simulink model "heli_q8lab2"  (R2020b)
settings: Solver=ode1  StartTime=0.0  StopTime=inf  FixedStep=0.002  RelTol=1e-3  EnableMultiTasking=on
PostLoadFcn:
  | qc_set_target_type(getConfigSet(bdroot, 'QUARC Default Target Configuration'));
values from neighbouring files (symbols this model uses):
  F = [0 0; 0 0]    [init_heli_3_10lab2integral.m]    (also in init_heli_3_10lab2nointegral.m = [K(1, 1) K(1, 3))
  Joystick_gain_x = 1    [init_heli_3_10lab2integral.m]    (also in init_heli_3_10lab2nointegral.m)
  Joystick_gain_y = -1    [init_heli_3_10lab2integral.m]    (also in init_heli_3_10lab2nointegral.m)
  K_pd = -(lambda_1 + lambda_2)/K1    [init_heli_3_10lab2integral.m]    (also in init_heli_3_10lab2nointegral.m)
  K_pp = (lambda_1*lambda_2)/K1    [init_heli_3_10lab2integral.m]    (also in init_heli_3_10lab2nointegral.m)
undefined symbols (not defined in the file or in its folder): HIL, K, qc_get_step_size
libraries: quarc_library x4
settings Model: SimulationMode=external  ExtModeTrigDuration=5000  Creator=Rchan  LastModifiedBy=arnstein
settings SolverCC: PositivePriorityOrder=on
settings DataIOCC: LimitDataPoints=on  SaveFormat=Array  SignalLoggingSaveFormat=ModelDataLogs  ReturnWorkspaceOutputs=off
settings OptimizationCC: ExpressionDepthLimit=2147483647  InitFltsAndDblsToZero=on  LifeSpan=inf
settings DebuggingCC: SaveWithParameterizedLinksMsg=none  UnderspecifiedInitializationDetection=Classic  MergeDetectMultiDrivingBlocksExec=none  SolverPrmCheckMsg=warning  MultiTaskDSMMsg=warning  MultiTaskCondExecSysMsg=none  FcnCallInpInsideContextMsg=warning  AllowSymbolicDim=off  StateNameClashWarn=warning  SFUnexpectedBacktrackingDiag=warning  SFNoUnconditionalDefaultTransitionDiag=warning  SFExecutionAtInitializationDiag=none  ArithmeticOperatorsInVariantConditions=warning
settings HardwareCC: ProdBitPerPointer=32  ProdBitPerSizeT=32  ProdBitPerPtrDiffT=32  ProdLargestAtomicFloat=None  ProdIntDivRoundTo=Undefined  ProdEndianess=Unspecified  ProdWordSize=32  ProdHWDeviceType=32-bit Generic
settings ModelReferenceCC: PropagateSignalLabelsOutOfModel=off
settings SFSimCC: SimUseLocalCustomCode=off  CustomCodeUndefinedFunction=UseInterfaceOnly
settings RTWCC: Description=QUARC Win64 Target  SystemTargetFile=quarc_win64.tlc  TemplateMakefile=quarc_default_tmf  RTWUseLocalCustomCode=off
settings CodeAppCC: StateflowObjectComments=on
settings GRTTargetCC: TargetLangStandard=C89/C90 (ANSI)  ParMdlRefBuildCompliant=off  CompOptLevelCompliant=off  CombineOutputUpdateFcns=off  MatFileLogging=off  GRTInterface=on  UseToolchainInfoCompliant=off  ExtMode=on  ExtModeMexFile=quarc_comm
settings ConfigComp: CovMetricSettings=de  CovSaveCumulativeToWorkspaceVar=on  CovSaveSingleToWorkspaceVar=on  CovExternalEMLEnable=off  CovSFcnEnable=off  CovBoundaryAbsTol=1.0e-5

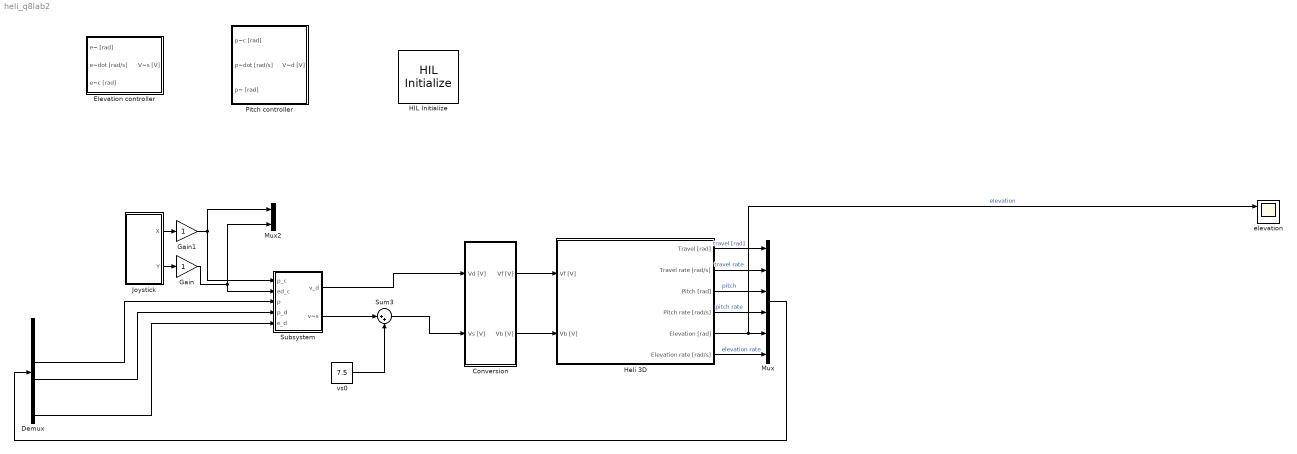
== system heli_q8lab2 ==
  Conversion : Subsystem
  Demux : Demux  Outputs=6
  Elevation controller : Subsystem
  Gain : Gain
  Gain1 : Gain
  HIL Initialize : quarc_library/Data Acquisition/Generic/Configuration/HIL Initialize  Priority=-99  object_name=HIL-1  board_type=q8_usb  board_number=0  board_options=update_rate=normal;decimation=1  exclusive=off  active=off  hardware_clocks=[0:2]  clock_modes=[]  initial_clock_frequencies=[]  set_clock_params_at_start=off  set_clock_params_at_switch_in=off  set_clock_frequencies_at_start=off  set_clock_frequencies_at_switch_in=off  analog_input_channels=[0:7]  analog_input_configurations=[]  analog_input_maximums=10  analog_input_minimums=-10  set_analog_input_params_at_start=on  set_analog_input_params_at_switch_in=off  analog_output_channels=[0:7]  analog_output_maximums=10  analog_output_minimums=-10  initial_analog_outputs=[0]  final_analog_outputs=[0]  watchdog_analog_outputs=0  set_analog_output_params_at_start=on  set_analog_output_params_at_switch_in=off  set_analog_outputs_at_start=on  set_analog_outputs_at_switch_in=off  set_analog_outputs_at_terminate=on  set_analog_outputs_at_switch_out=off  set_analog_outputs_on_watchdog=off  digital_input_channels=[]  digital_output_channels=[]  digital_output_configuration=[]  initial_digital_outputs=[1]  final_digital_outputs=[1]  watchdog_digital_outputs=[1]  set_digital_output_params_at_start=off  set_digital_output_params_at_switch_in=off  set_digital_outputs_at_start=on  set_digital_outputs_at_switch_in=off  set_digital_outputs_at_terminate=on  set_digital_outputs_at_switch_out=off  set_digital_outputs_on_watchdog=off  encoder_channels=[0:7]  quadrature=[4]  encoder_filter_frequency=[]  initial_encoder_counts=[0]  set_encoder_params_at_start=on  set_encoder_params_at_switch_in=off  set_encoder_counts_at_start=on  set_encoder_counts_at_switch_in=off  pwm_channels=[0:7]  pwm_modes=0  pwm_frequency=99.532799999999995e6/4095  pwm_configuration=[0]  pwm_alignment=[0]  pwm_polarity=[1]  pwm_leading_deadband=[0]  pwm_trailing_deadband=[0]  initial_pwm_outputs=[0]  final_pwm_outputs=[0]  watchdog_pwm_outputs=[0]  set_pwm_params_at_start=on  set_pwm_params_at_switch_in=off  set_pwm_outputs_at_start=on  set_pwm_outputs_at_switch_in=off  set_pwm_outputs_at_terminate=on  set_pwm_outputs_at_switch_out=off  set_pwm_outputs_on_watchdog=off  other_output_channels=[]  initial_other_outputs=[]  final_other_outputs=[]  watchdog_other_outputs=[]  set_other_outputs_at_start=off  set_other_outputs_at_switch_in=off  set_other_outputs_at_terminate=off  set_other_outputs_at_switch_out=off  set_other_outputs_on_watchdog=off
  Heli 3D : Subsystem
  Joystick : Subsystem
  Mux : Mux  Inputs=6
  Mux2 : Mux  Inputs=2
  Pitch controller : Subsystem
  Subsystem : Subsystem
  Sum3 : Sum  Inputs=|++
  elevation : Scope  NumInputPorts=2
  vs0 : Constant  Value=7.5
  wires:
  Conversion/2(Vb [V]) -> Heli 3D/2(Vb [V])
  Conversion/1(Vf [V]) -> Heli 3D/1(Vf [V])
  Heli 3D/1(Travel [rad]) -> Mux/1  "travel [rad]"
  Heli 3D/2(Travel rate [rad/s]) -> Mux/2  "travel rate"
  Heli 3D/3(Pitch [rad]) -> Mux/3  "pitch"
  Heli 3D/4(Pitch rate [rad/s]) -> Mux/4  "pitch rate"
  Heli 3D/5(Elevation [rad]) -> elevation/1, Mux/5  "elevation"
  Heli 3D/6(Elevation rate [rad/s]) -> Mux/6  "elevation rate"
  Joystick/1(X) -> Gain1/1
  Joystick/2(Y) -> Gain/1
  Gain/1 -> Mux2/2, Subsystem/2(ed_c)
  Gain1/1 -> Mux2/1, Subsystem/1(p_c)
  Subsystem/1(v_d) -> Conversion/1(Vd [V])
  Subsystem/2(v~s) -> Sum3/1
  Sum3/1 -> Conversion/2(Vs [V])
  vs0/1 -> Sum3/2
  Demux/3 -> Subsystem/3(p)
  Demux/4 -> Subsystem/4(p_d)
  Demux/6 -> Subsystem/5(e_d)
  Mux/1 -> Demux/1

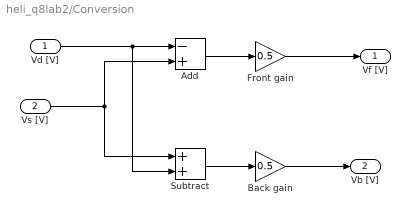
== system heli_q8lab2/Conversion ==
  Vd [V] : Inport
  Vs [V] : Inport  Port=2
  Add : Sum  Inputs=-+
  Back gain : Gain  Gain=0.5
  Front gain : Gain  Gain=0.5
  Subtract : Sum
  Vf [V] : Outport
  Vb [V] : Outport  Port=2
  wires:
  Vd [V]/1 -> Subtract/2, Add/1
  Vs [V]/1 -> Subtract/1, Add/2
  Subtract/1 -> Back gain/1
  Back gain/1 -> Vb [V]/1
  Add/1 -> Front gain/1
  Front gain/1 -> Vf [V]/1

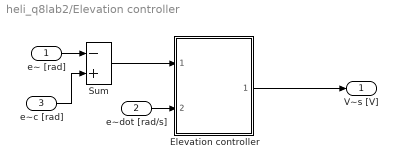
== system heli_q8lab2/Elevation controller ==
  e~ [rad] : Inport
  e~dot [rad/s] : Inport  Port=2
  e~c [rad] : Inport  Port=3
  Elevation controller : Subsystem
  Sum : Sum  Inputs=-+  InputSameDT=on  SaturateOnIntegerOverflow=on  OutDataTypeStr=Inherit: Same as first input
  V~s [V] : Outport  InitialOutput=0
  wires:
  Sum/1 -> Elevation controller/1(e~ [rad])
  Elevation controller/1(V~_s [V]) -> V~s [V]/1
  e~ [rad]/1 -> Sum/1
  e~dot [rad/s]/1 -> Elevation controller/2(e~_dot [rad/s])
  e~c [rad]/1 -> Sum/2

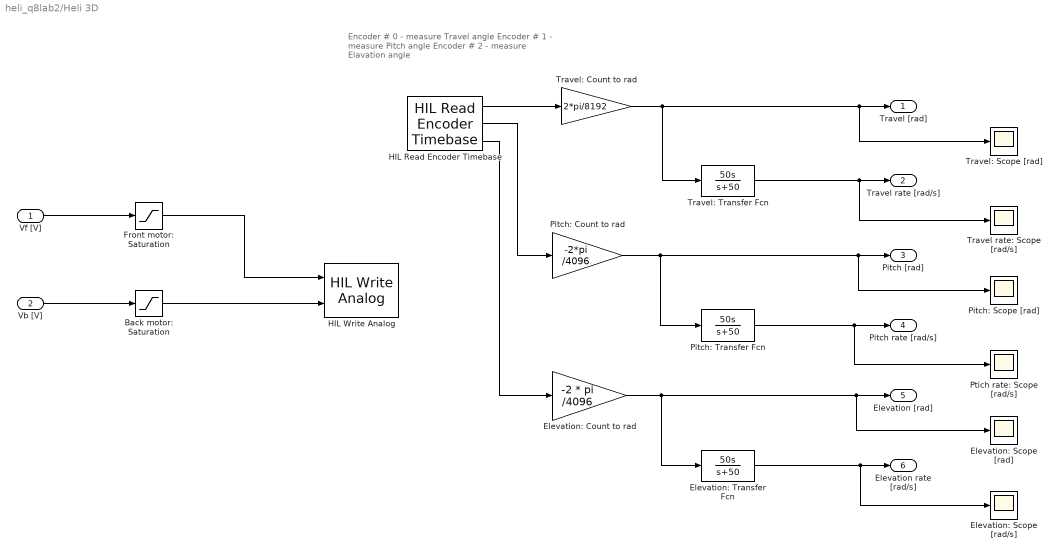
== system heli_q8lab2/Heli 3D ==
  note: Encoder # 0 - measure Travel angle
      | Encoder # 1 - measure Pitch angle
      | Encoder # 2 - measure Elavation angle
  Vf [V] : Inport
  Vb [V] : Inport  Port=2
  Back motor: Saturation : Saturate  UpperLimit=5  LowerLimit=-5
  Elevation: Count to rad : Gain  Gain=-2 * pi /4096
  Elevation: Scope [rad/s] : Scope
  Elevation: Scope [rad] : Scope
  Elevation: Transfer Fcn : TransferFcn  Numerator=[50 0]  Denominator=[1 50]
  Front motor: Saturation : Saturate  UpperLimit=5  LowerLimit=-5
  HIL Read Encoder Timebase : quarc_library/Data Acquisition/Generic/Timebases/HIL Read Encoder Timebase  object_name=HIL-1  clock=0  channels=[0:2]  active=on  vector_output=off  data_type_mode=Inherit via back propagation  data_type=double  overflow_mode=Error on overflow  samples_in_buffer=max(ceil(1/qc_get_step_size), 1)
  HIL Write Analog : quarc_library/Data Acquisition/Generic/Immediate I//O/HIL Write Analog  object_name=HIL-1  channels=[0:1]  sample_time=-1  active=off  vector_input=off
  Pitch: Count to rad : Gain  Gain=-2*pi /4096
  Pitch: Scope [rad] : Scope
  Pitch: Transfer Fcn : TransferFcn  Numerator=[50 0]  Denominator=[1 50]
  Ptich rate: Scope [rad/s] : Scope
  Travel rate: Scope [rad/s] : Scope
  Travel: Count to rad : Gain  Gain=2*pi/8192
  Travel: Scope [rad] : Scope
  Travel: Transfer Fcn : TransferFcn  Numerator=[50 0]  Denominator=[1 50]
  Travel [rad] : Outport
  Travel rate [rad/s] : Outport  Port=2
  Pitch [rad] : Outport  Port=3
  Pitch rate [rad/s] : Outport  Port=4
  Elevation [rad] : Outport  Port=5
  Elevation rate [rad/s] : Outport  Port=6
  wires:
  HIL Read Encoder Timebase/1 -> Travel: Count to rad/1
  HIL Read Encoder Timebase/2 -> Pitch: Count to rad/1
  HIL Read Encoder Timebase/3 -> Elevation: Count to rad/1
  Travel: Count to rad/1 -> Travel: Scope [rad]/1, Travel [rad]/1, Travel: Transfer Fcn/1
  Travel: Transfer Fcn/1 -> Travel rate: Scope [rad/s]/1, Travel rate [rad/s]/1
  Pitch: Count to rad/1 -> Pitch: Transfer Fcn/1, Pitch: Scope [rad]/1, Pitch [rad]/1
  Pitch: Transfer Fcn/1 -> Ptich rate: Scope [rad/s]/1, Pitch rate [rad/s]/1
  Elevation: Count to rad/1 -> Elevation: Transfer Fcn/1, Elevation: Scope [rad]/1, Elevation [rad]/1
  Elevation: Transfer Fcn/1 -> Elevation: Scope [rad/s]/1, Elevation rate [rad/s]/1
  Vf [V]/1 -> Front motor: Saturation/1
  Vb [V]/1 -> Back motor: Saturation/1
  Front motor: Saturation/1 -> HIL Write Analog/1
  Back motor: Saturation/1 -> HIL Write Analog/2

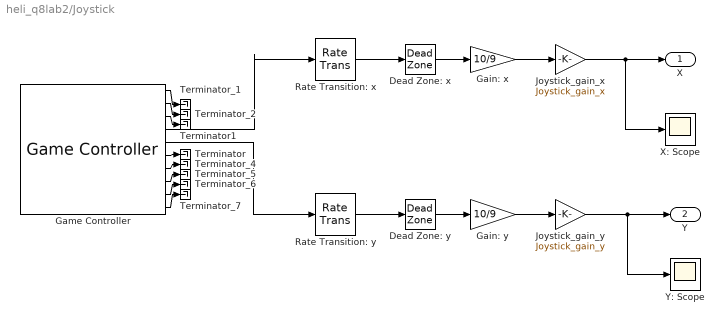
== system heli_q8lab2/Joystick ==
  Dead Zone: x : DeadZone  LowerValue=-0.1  UpperValue=0.1  SaturateOnIntegerOverflow=on
  Dead Zone: y : DeadZone  LowerValue=-0.1  UpperValue=0.1  SaturateOnIntegerOverflow=on
  Gain: x : Gain  Gain=10/9
  Gain: y : Gain  Gain=10/9
  Game Controller : quarc_library/Devices/Peripherals/Target/Game Controller  controller=1  buffer_size=12  deadzone=[]  saturation=[]  sample_time=max(qc_get_step_size, 0.01)  auto_center=off  enabled=on
      settings: SourceProductName=QUARC Targets
  Joystick_gain_x : Gain  Gain=Joystick_gain_x
  Joystick_gain_y : Gain  Gain=Joystick_gain_y
  Rate Transition: x : RateTransition
  Rate Transition: y : RateTransition
  Terminator : Terminator
  Terminator1 : Terminator
  Terminator_{1..2,4..7} (6 alike) : Terminator
  X: Scope : Scope
  Y: Scope : Scope
  X : Outport
  Y : Outport  Port=2
  wires:
  Rate Transition: y/1 -> Dead Zone: y/1
  Rate Transition: x/1 -> Dead Zone: x/1
  Game Controller/5 -> Rate Transition: y/1
  Game Controller/4 -> Rate Transition: x/1
  Game Controller/1 -> Terminator_1/1
  Game Controller/2 -> Terminator_2/1
  Game Controller/7 -> Terminator_4/1
  Game Controller/8 -> Terminator_5/1
  Game Controller/9 -> Terminator_6/1
  Game Controller/10 -> Terminator_7/1
  Game Controller/3 -> Terminator1/1
  Game Controller/6 -> Terminator/1
  Dead Zone: x/1 -> Gain: x/1
  Dead Zone: y/1 -> Gain: y/1
  Gain: x/1 -> Joystick_gain_x/1
  Gain: y/1 -> Joystick_gain_y/1
  Joystick_gain_x/1 -> X/1, X: Scope/1
  Joystick_gain_y/1 -> Y: Scope/1, Y/1

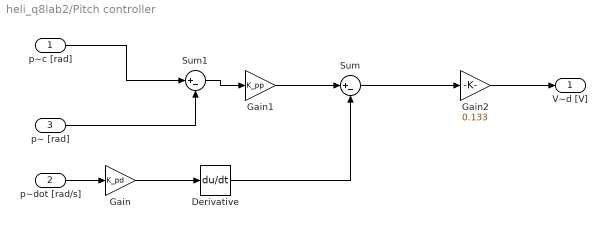
== system heli_q8lab2/Pitch controller ==
  p~c [rad] : Inport
  p~dot [rad/s] : Inport  Port=2
  p~ [rad] : Inport  Port=3
  Derivative : Derivative
  Gain : Gain  Gain=K_pd
  Gain1 : Gain  Gain=K_pp
  Gain2 : Gain  Gain=0.133
  Sum : Sum  Inputs=|+-
  Sum1 : Sum  Inputs=|+-
  V~d [V] : Outport  InitialOutput=0
  wires:
  p~dot [rad/s]/1 -> Gain/1
  Gain/1 -> Derivative/1
  Derivative/1 -> Sum/2
  p~c [rad]/1 -> Sum1/1
  p~ [rad]/1 -> Sum1/2
  Sum1/1 -> Gain1/1
  Gain1/1 -> Sum/1
  Sum/1 -> Gain2/1
  Gain2/1 -> V~d [V]/1

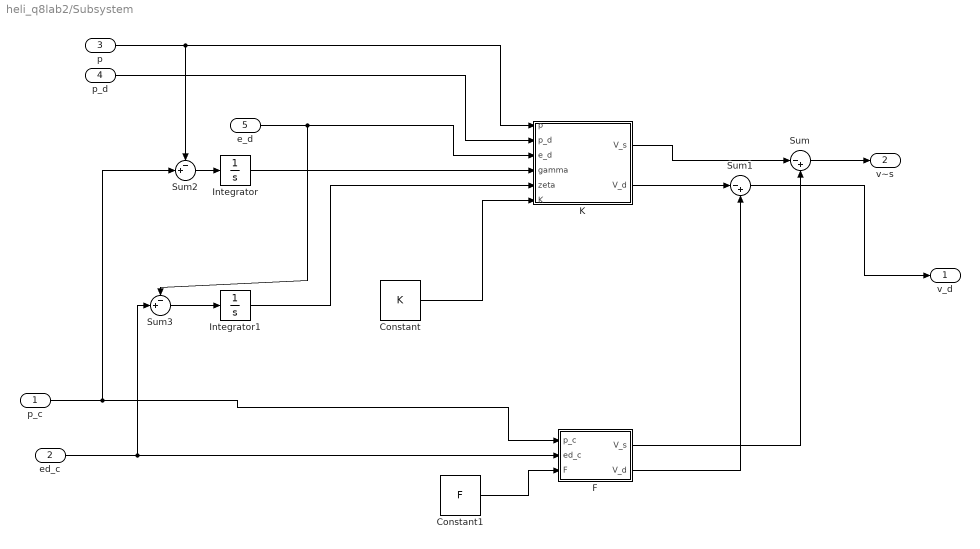
== system heli_q8lab2/Subsystem ==
  p_c : Inport
  ed_c : Inport  Port=2
  p : Inport  Port=3
  p_d : Inport  Port=4
  e_d : Inport  Port=5
  Constant : Constant  Value=K
  Constant1 : Constant  Value=F
  F : MATLAB Function  TreatAsAtomicUnit=on
  Integrator : Integrator
  Integrator1 : Integrator
  K : MATLAB Function  TreatAsAtomicUnit=on
  Sum : Sum  Inputs=|-+
  Sum1 : Sum  Inputs=|-+
  Sum2 : Sum  Inputs=-+|
  Sum3 : Sum  Inputs=-+|
  v_d : Outport
  v~s : Outport  Port=2
  wires:
  p/1 -> Sum2/1, K/1(p)
  p_d/1 -> K/2(p_d)
  e_d/1 -> Sum3/1, K/3(e_d)
  Constant/1 -> K/6(K)
  Constant1/1 -> F/3(F)
  p_c/1 -> Sum2/2, F/1(p_c)
  ed_c/1 -> Sum3/2, F/2(ed_c)
  K/1(V_s) -> Sum/1
  Sum/1 -> v~s/1
  K/2(V_d) -> Sum1/1
  F/1(V_s) -> Sum/2
  F/2(V_d) -> Sum1/2
  Sum1/1 -> v_d/1
  Integrator/1 -> K/4(gamma)
  Integrator1/1 -> K/5(zeta)
  Sum2/1 -> Integrator/1
  Sum3/1 -> Integrator1/1

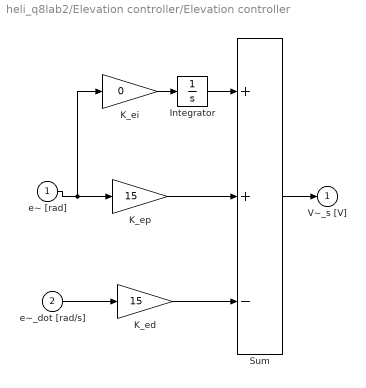
== system heli_q8lab2/Elevation controller/Elevation controller ==
  e~ [rad] : Inport
  e~_dot [rad/s] : Inport  Port=2
  Integrator : Integrator  LimitOutput=on
  K_ed : Gain  Gain=15  SaturateOnIntegerOverflow=on  OutDataTypeStr=Inherit: Same as input  ParamDataTypeStr=Inherit: Same as input
  K_ei : Gain  Gain=0  SaturateOnIntegerOverflow=on  OutDataTypeStr=Inherit: Same as input  ParamDataTypeStr=Inherit: Same as input
  K_ep : Gain  Gain=15  SaturateOnIntegerOverflow=on  OutDataTypeStr=Inherit: Same as input  ParamDataTypeStr=Inherit: Same as input
  Sum : Sum  Inputs=++-  InputSameDT=on  SaturateOnIntegerOverflow=on  OutDataTypeStr=Inherit: Same as first input
  V~_s [V] : Outport  InitialOutput=0
  wires:
  K_ei/1 -> Integrator/1
  Integrator/1 -> Sum/1
  Sum/1 -> V~_s [V]/1
  e~_dot [rad/s]/1 -> K_ed/1
  K_ed/1 -> Sum/3
  K_ep/1 -> Sum/2
  e~ [rad]/1 -> K_ep/1, K_ei/1

== matlab function heli_q8lab2/Subsystem/F ==
  data: p_c input; V_s output; V_d output; ed_c input; F input
function [V_s, V_d] = fcn(p_c, ed_c, F)
M = (F*[p_c, ed_c].');
V_s = M(1, :);
V_d = M(2, :);
end

== matlab function heli_q8lab2/Subsystem/K ==
  data: p input; V_s output; V_d output; p_d input; e_d input; gamma input; zeta input; K input
function [V_s, V_d] = fcn(p, p_d, e_d, gamma, zeta, K)
M = (K*[p, p_d, e_d, gamma, zeta].');
V_s = M(1, :);
V_d = M(2, :);
end
